simulink model "lcc_closed_loop"  (R2026b)
settings: Solver=ode4  StopTime=60  FixedStep=0.005
values from neighbouring files (symbols this model uses):
  SCN = struct("speed", v, "wheelbase", opts.Wheelbase, "trailer", P.trailer_connected, "enable", true,      "base", struct("lookahead_m", 6, "lookahead_time_s", 0.7, "window", opts.Window))    [lcc_scenario_input.m]
settings Model: Creator=kikiw  LastModifiedBy=kikiw
settings SolverCC: AutoInsertRateTranBlk=on
settings DataIOCC: SignalLogging=off

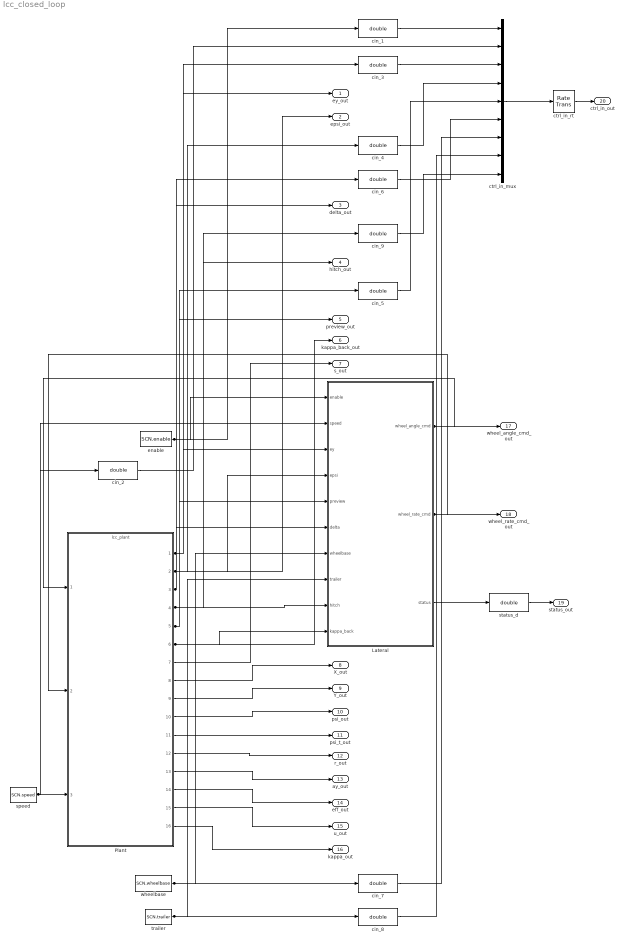
== system lcc_closed_loop ==
  Lateral : Subsystem  Variant=on
  Plant : ModelReference  ModelNameDialog=lcc_plant  SimulationMode=Normal  ModelReferenceVersion=1.1
  cin_{1..9} (9 alike) : DataTypeConversion  OutDataTypeStr=double  SaturateOnIntegerOverflow=off  RndMeth=Floor
  ctrl_in_mux : Mux  Inputs=9
  ctrl_in_rt : RateTransition  OutPortSampleTime=0.02
  enable : Constant  Value=SCN.enable  OutDataTypeStr=boolean  SampleTime=0.02
  speed : Constant  Value=SCN.speed
  status_d : DataTypeConversion  OutDataTypeStr=double  SaturateOnIntegerOverflow=off  RndMeth=Floor
  trailer : Constant  Value=SCN.trailer  OutDataTypeStr=boolean  SampleTime=0.02
  wheelbase : Constant  Value=SCN.wheelbase  SampleTime=0.02
  ey_out : Outport
  epsi_out : Outport  Port=2
  delta_out : Outport  Port=3
  hitch_out : Outport  Port=4
  preview_out : Outport  Port=5
  kappa_back_out : Outport  Port=6
  s_out : Outport  Port=7
  X_out : Outport  Port=8
  Y_out : Outport  Port=9
  psi_out : Outport  Port=10
  psi_t_out : Outport  Port=11
  r_out : Outport  Port=12
  ay_out : Outport  Port=13
  eff_out : Outport  Port=14
  u_out : Outport  Port=15
  kappa_out : Outport  Port=16
  wheel_angle_cmd_out : Outport  Port=17
  wheel_rate_cmd_out : Outport  Port=18
  status_out : Outport  Port=19
  ctrl_in_out : Outport  Port=20
  wires:
  wheelbase/1 -> cin_7/1, Lateral/7(wheelbase)
  speed/1 -> Lateral/2(speed), Plant/3, cin_2/1
  enable/1 -> Lateral/1(enable), cin_1/1
  cin_2/1 -> ctrl_in_mux/2
  Plant/2 -> Lateral/4(epsi), epsi_out/1, cin_4/1
  Plant/1 -> Lateral/3(ey), ey_out/1, cin_3/1
  Plant/9 -> Y_out/1
  Plant/7 -> s_out/1
  Plant/3 -> Lateral/6(delta), delta_out/1, cin_6/1
  Plant/5 -> preview_out/1, cin_5/1, Lateral/5(preview)
  Lateral/2(wheel_rate_cmd) -> Plant/2, wheel_rate_cmd_out/1
  Plant/10 -> psi_out/1
  Plant/8 -> X_out/1
  Plant/6 -> Lateral/10(kappa_back), kappa_back_out/1
  Plant/4 -> Lateral/9(hitch), hitch_out/1, cin_9/1
  Plant/15 -> u_out/1
  Plant/13 -> ay_out/1
  Plant/11 -> psi_t_out/1
  Plant/16 -> kappa_out/1
  Plant/14 -> eff_out/1
  Plant/12 -> r_out/1
  trailer/1 -> Lateral/8(trailer), cin_8/1
  cin_1/1 -> ctrl_in_mux/1
  cin_3/1 -> ctrl_in_mux/3
  cin_4/1 -> ctrl_in_mux/4
  cin_6/1 -> ctrl_in_mux/6
  ctrl_in_mux/1 -> ctrl_in_rt/1
  Lateral/1(wheel_angle_cmd) -> Plant/1, wheel_angle_cmd_out/1
  cin_9/1 -> ctrl_in_mux/9
  cin_5/1 -> ctrl_in_mux/5
  ctrl_in_rt/1 -> ctrl_in_out/1
  Lateral/3(status) -> status_d/1
  cin_7/1 -> ctrl_in_mux/7
  cin_8/1 -> ctrl_in_mux/8
  status_d/1 -> status_out/1

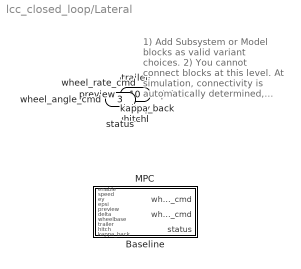
== system lcc_closed_loop/Lateral ==
  note: 1) Add Subsystem or Model blocks as valid variant choices.
      | 2) You cannot connect blocks at this level. At simulation, connectivity is automatically
      | determined, based on the active variant and port name matching.
  enable : Inport
  speed : Inport  Port=2
  ey : Inport  Port=3
  epsi : Inport  Port=4
  preview : Inport  Port=5
  delta : Inport  Port=6
  wheelbase : Inport  Port=7
  trailer : Inport  Port=8
  hitch : Inport  Port=9
  kappa_back : Inport  Port=10
  Baseline : Subsystem  VariantControl=LCC_CTRL == 1
  MPC : Subsystem  VariantControl=LCC_CTRL == 2
  wheel_angle_cmd : Outport
  wheel_rate_cmd : Outport  Port=2
  status : Outport  Port=3

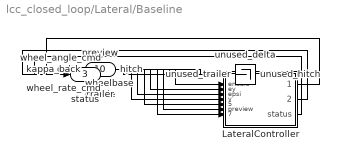
== system lcc_closed_loop/Lateral/Baseline ==
  enable : Inport
  speed : Inport  Port=2
  ey : Inport  Port=3
  epsi : Inport  Port=4
  preview : Inport  Port=5
  delta : Inport  Port=6
  wheelbase : Inport  Port=7
  trailer : Inport  Port=8
  hitch : Inport  Port=9
  kappa_back : Inport  Port=10
  LateralController : MATLAB Function  TreatAsAtomicUnit=on  SystemSampleTime=0.02
  unused_delta : Terminator
  unused_hitch : Terminator
  unused_trailer : Terminator
  wheel_angle_cmd : Outport
  wheel_rate_cmd : Outport  Port=2
  status : Outport  Port=3
  wires:
  enable/1 -> LateralController/1(enable)
  ey/1 -> LateralController/2(ey)
  epsi/1 -> LateralController/3(epsi)
  speed/1 -> LateralController/4(v)
  wheelbase/1 -> LateralController/5(wheelbase)
  preview/1 -> LateralController/6(preview)
  kappa_back/1 -> LateralController/7(kappa_back)
  LateralController/1(wheel_angle) -> wheel_angle_cmd/1
  LateralController/2(wheel_rate) -> wheel_rate_cmd/1
  LateralController/3(status) -> status/1
  delta/1 -> unused_delta/1
  trailer/1 -> unused_trailer/1
  hitch/1 -> unused_hitch/1

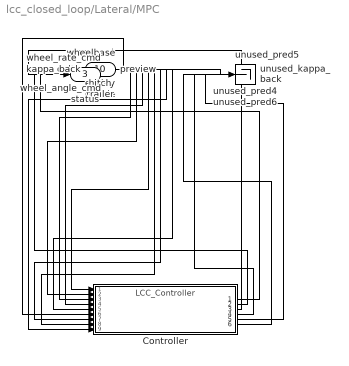
== system lcc_closed_loop/Lateral/MPC ==
  enable : Inport
  speed : Inport  Port=2
  ey : Inport  Port=3
  epsi : Inport  Port=4
  preview : Inport  Port=5
  delta : Inport  Port=6
  wheelbase : Inport  Port=7
  trailer : Inport  Port=8
  hitch : Inport  Port=9
  kappa_back : Inport  Port=10
  Controller : ModelReference  ModelNameDialog=LCC_Controller  SimulationMode=Normal  ModelReferenceVersion=1.1
  unused_kappa_back : Terminator
  unused_pred4 : Terminator
  unused_pred5 : Terminator
  unused_pred6 : Terminator
  wheel_angle_cmd : Outport
  wheel_rate_cmd : Outport  Port=2
  status : Outport  Port=3
  wires:
  enable/1 -> Controller/1
  speed/1 -> Controller/2
  ey/1 -> Controller/3
  epsi/1 -> Controller/4
  preview/1 -> Controller/5
  delta/1 -> Controller/6
  wheelbase/1 -> Controller/7
  trailer/1 -> Controller/8
  hitch/1 -> Controller/9
  Controller/1 -> wheel_angle_cmd/1
  Controller/2 -> wheel_rate_cmd/1
  Controller/3 -> status/1
  Controller/4 -> unused_pred4/1
  Controller/5 -> unused_pred5/1
  Controller/6 -> unused_pred6/1
  kappa_back/1 -> unused_kappa_back/1

== matlab function lcc_closed_loop/Lateral/Baseline/LateralController ==
  data: enable input; wheel_angle output; ey input; epsi input; v input; wheelbase input; preview input; kappa_back input; wheel_rate output; status output; SCN parameter
function [wheel_angle, wheel_rate, status] = LateralController(enable, ey, epsi, v, wheelbase, preview, kappa_back, SCN)
% lateral_controller.hpp (LateralController::update), 50 Hz
[wheel_angle, wheel_rate] = lcc_baseline(ey, epsi, v, wheelbase, preview, kappa_back, SCN.base);
status = uint8(enable);
